simulink model "nms_sim_2D_cost"  (R2024b)
settings: Solver=ode15s  StartTime=0.0  StopTime=t_sim  MaxStep=dt_max  EnableMultiTasking=on
values from neighbouring files (symbols this model uses):
  a_BFSH = param_ctrl(35)*1    [setCtrlPar_optim_CPGreflex2001_2D.m]
  a_GAS = param_ctrl(37)*1    [setCtrlPar_optim_CPGreflex2001_2D.m]
  a_GLU = param_ctrl(31)*1    [setCtrlPar_optim_CPGreflex2001_2D.m]
  a_HAM = param_ctrl(33)*1    [setCtrlPar_optim_CPGreflex2001_2D.m]
  a_HFL = param_ctrl(32)*1    [setCtrlPar_optim_CPGreflex2001_2D.m]
  a_RF = param_ctrl(34)*1    [setCtrlPar_optim_CPGreflex2001_2D.m]
  a_SOL = param_ctrl(38)*1    [setCtrlPar_optim_CPGreflex2001_2D.m]
  a_TA = param_ctrl(39)*1    [setCtrlPar_optim_CPGreflex2001_2D.m]
  a_VAS = param_ctrl(36)*1    [setCtrlPar_optim_CPGreflex2001_2D.m]
  ai = param_ctrl(96)*2.0    [setCtrlPar_optim_CPGreflex2001_2D.m]
  b_BFSH = param_ctrl(52)*.51    [setCtrlPar_optim_CPGreflex2001_2D.m]
  b_BFSHGAS = param_ctrl(55)*.51    [setCtrlPar_optim_CPGreflex2001_2D.m]
  b_BFSHHAM = param_ctrl(54)*.51    [setCtrlPar_optim_CPGreflex2001_2D.m]
  b_BFSHVAS = param_ctrl(53)*.51    [setCtrlPar_optim_CPGreflex2001_2D.m]
  b_GAS = param_ctrl(59)*.51    [setCtrlPar_optim_CPGreflex2001_2D.m]
  b_GASBFSH = param_ctrl(60)*.51    [setCtrlPar_optim_CPGreflex2001_2D.m]
  b_GASSOL = param_ctrl(61)*.51    [setCtrlPar_optim_CPGreflex2001_2D.m]
  b_GLU = param_ctrl(40)*.51    [setCtrlPar_optim_CPGreflex2001_2D.m]
  b_GLUHAM = param_ctrl(42)*.51    [setCtrlPar_optim_CPGreflex2001_2D.m]
  b_GLUHFL = param_ctrl(41)*.51    [setCtrlPar_optim_CPGreflex2001_2D.m]
  b_HAM = param_ctrl(46)*.51    [setCtrlPar_optim_CPGreflex2001_2D.m]
  b_HAMBFSH = param_ctrl(48)*.51    [setCtrlPar_optim_CPGreflex2001_2D.m]
  b_HAMGLU = param_ctrl(47)*.51    [setCtrlPar_optim_CPGreflex2001_2D.m]
  b_HFL = param_ctrl(43)*.51    [setCtrlPar_optim_CPGreflex2001_2D.m]
  b_HFLGLU = param_ctrl(44)*.51    [setCtrlPar_optim_CPGreflex2001_2D.m]
  b_HFLRF = param_ctrl(45)*.51    [setCtrlPar_optim_CPGreflex2001_2D.m]
  b_RF = param_ctrl(49)*.51    [setCtrlPar_optim_CPGreflex2001_2D.m]
  b_RFHFL = param_ctrl(50)*.51    [setCtrlPar_optim_CPGreflex2001_2D.m]
  b_RFVAS = param_ctrl(51)*.51    [setCtrlPar_optim_CPGreflex2001_2D.m]
  b_SOL = param_ctrl(62)*.51    [setCtrlPar_optim_CPGreflex2001_2D.m]
  b_SOLGAS = param_ctrl(64)*.51    [setCtrlPar_optim_CPGreflex2001_2D.m]
  b_SOLTA = param_ctrl(63)*.51    [setCtrlPar_optim_CPGreflex2001_2D.m]
  b_TA = param_ctrl(65)*.51    [setCtrlPar_optim_CPGreflex2001_2D.m]
  b_TASOL = param_ctrl(66)*.51    [setCtrlPar_optim_CPGreflex2001_2D.m]
  b_VAS = param_ctrl(56)*.51    [setCtrlPar_optim_CPGreflex2001_2D.m]
  b_VASBFSH = param_ctrl(57)*.51    [setCtrlPar_optim_CPGreflex2001_2D.m]
  b_VASRF = param_ctrl(58)*.51    [setCtrlPar_optim_CPGreflex2001_2D.m]
  bias = param_ctrl(97)*2.5    [setCtrlPar_optim_CPGreflex2001_2D.m]
  c = 0.05    [nms_MS_2D_scaled.m]
  c_jointstop = 0.3 / (pi/180)    (= 17.1887338539)    [nms_MS_2D_scaled.m]
  D12_F = 0.16    *scaleL_JPhys    [nms_MechInit_2D_scaleSkel.m]
  D12_S = 0.2460	*sub_height    [nms_MechInit_2D_scaleSkel.m]
  D12_T = 0.2450  *sub_height    [nms_MechInit_2D_scaleSkel.m]
  D12y_F = 0.039  *sub_height    [nms_MechInit_2D_scaleSkel.m]
  D12z_HAT = 0.1    [nms_MS_2D_scaled.m]
  D13_F = 0.20    *scaleL_JPhys    [nms_MechInit_2D_scaleSkel.m]
  D1G_F = 0.14    *scaleL_JPhys    [nms_MechInit_2D_scaleSkel.m]
  D1G_HAT = 0.35  *scaleL_JPhys    [nms_MechInit_2D_scaleSkel.m]
  D1G_S = (0.3 - D12y_F/4)	*scaleL_JPhys    [nms_MechInit_2D_scaleSkel.m]
  D1G_T = (0.3 - D12y_F/4)	*scaleL_JPhys    [nms_MechInit_2D_scaleSkel.m]
  D1Gy_F = D12y_F*D1G_F/D12_F    (= 0.07)    [nms_MechInit_2D_scaleSkel.m]
  d_BFSH = param_ctrl(26)*1    [setCtrlPar_optim_CPGreflex2001_2D.m]
  d_GAS = param_ctrl(28)*1    [setCtrlPar_optim_CPGreflex2001_2D.m]
  d_GLU = param_ctrl(22)*1    [setCtrlPar_optim_CPGreflex2001_2D.m]
  d_HAM = param_ctrl(24)*1    [setCtrlPar_optim_CPGreflex2001_2D.m]
  d_HFL = param_ctrl(23)*1    [setCtrlPar_optim_CPGreflex2001_2D.m]
  d_RF = param_ctrl(25)*1    [setCtrlPar_optim_CPGreflex2001_2D.m]
  d_SOL = param_ctrl(29)*1    [setCtrlPar_optim_CPGreflex2001_2D.m]
  d_TA = param_ctrl(30)*1    [setCtrlPar_optim_CPGreflex2001_2D.m]
  d_VAS = param_ctrl(27)*1    [setCtrlPar_optim_CPGreflex2001_2D.m]
  DeltaThRef = 5e-3    (= 0.005)    [nms_MS_2D_scaled.m]
  dloptBFSH = 3.0    (= 3)    [setCtrlPar_optim_CPGreflex2001_2D.m]
  dloptGAS = 3.0    (= 3)    [setCtrlPar_optim_CPGreflex2001_2D.m]
  dloptGLU = 3.0    (= 3)    [setCtrlPar_optim_CPGreflex2001_2D.m]
  dloptHAM = 3.0    (= 3)    [setCtrlPar_optim_CPGreflex2001_2D.m]
  dloptHFL = 3.0    (= 3)    [setCtrlPar_optim_CPGreflex2001_2D.m]
  dloptRF = 3.0    (= 3)    [setCtrlPar_optim_CPGreflex2001_2D.m]
  dloptSOL = 3.0    (= 3)    [setCtrlPar_optim_CPGreflex2001_2D.m]
  dloptTA = 3.0    (= 3)    [setCtrlPar_optim_CPGreflex2001_2D.m]
  dloptVAS = 3.0    (= 3)    [setCtrlPar_optim_CPGreflex2001_2D.m]
  ec_BFSH = param_ctrl(80)*0.15    [setCtrlPar_optim_CPGreflex2001_2D.m]
  ec_GAS = param_ctrl(82)*0.15    [setCtrlPar_optim_CPGreflex2001_2D.m]
  ec_GLU = param_ctrl(76)*0.15    [setCtrlPar_optim_CPGreflex2001_2D.m]
  ec_HAM = param_ctrl(78)*0.15    [setCtrlPar_optim_CPGreflex2001_2D.m]
  ec_HFL = param_ctrl(77)*0.15    [setCtrlPar_optim_CPGreflex2001_2D.m]
  ec_RF = param_ctrl(79)*0.15    [setCtrlPar_optim_CPGreflex2001_2D.m]
  ec_TA = param_ctrl(84)*0.15    [setCtrlPar_optim_CPGreflex2001_2D.m]
  ec_VAS = param_ctrl(81)*0.15    [setCtrlPar_optim_CPGreflex2001_2D.m]
  eref = 0.04    [nms_MS_2D_scaled.m]
  eref_GAS = 0.1    [nms_MS_2D_scaled.m]
  eref_SOL = 0.1    [nms_MS_2D_scaled.m]
  es_BFSH = param_ctrl(89)*0.15    [setCtrlPar_optim_CPGreflex2001_2D.m]
  es_GAS = param_ctrl(91)*0.15    [setCtrlPar_optim_CPGreflex2001_2D.m]
  es_GLU = param_ctrl(85)*0.15    [setCtrlPar_optim_CPGreflex2001_2D.m]
  es_HAM = param_ctrl(87)*0.15    [setCtrlPar_optim_CPGreflex2001_2D.m]
  es_HFL = param_ctrl(86)*0.15    [setCtrlPar_optim_CPGreflex2001_2D.m]
  es_RF = param_ctrl(88)*0.15    [setCtrlPar_optim_CPGreflex2001_2D.m]
  es_TA = param_ctrl(93)*0.15    [setCtrlPar_optim_CPGreflex2001_2D.m]
  es_VAS = param_ctrl(90)*0.15    [setCtrlPar_optim_CPGreflex2001_2D.m]
  FmaxBFSH = 350    [nms_MS_2D_scaled.m]
  FmaxGAS = 2000    [nms_MS_2D_scaled.m]
  FmaxGLU = 4000    [nms_MS_2D_scaled.m]
  FmaxHAM = 2000    [nms_MS_2D_scaled.m]
  FmaxHFL = 2000    [nms_MS_2D_scaled.m]
  FmaxRF = 850    [nms_MS_2D_scaled.m]
  FmaxSOL = 4000    [nms_MS_2D_scaled.m]
  FmaxTA = 800    [nms_MS_2D_scaled.m]
  FmaxVAS = 5000    [nms_MS_2D_scaled.m]
  g = 9.81    [nms_MS_2D_scaled.m]
  gamma_4 = param_ctrl(11) * 1.7    [setCtrlPar_optim_CPGreflexsynergy2023_2D.m]
  h_BFSH = param_ctrl(71)*.1    [setCtrlPar_optim_CPGreflex2001_2D.m]
  h_GAS = param_ctrl(73)*.1    [setCtrlPar_optim_CPGreflex2001_2D.m]
  h_GLU = param_ctrl(67)*.1    [setCtrlPar_optim_CPGreflex2001_2D.m]
  h_HAM = param_ctrl(69)*.1    [setCtrlPar_optim_CPGreflex2001_2D.m]
  h_HFL = param_ctrl(68)*.1    [setCtrlPar_optim_CPGreflex2001_2D.m]
  h_RF = param_ctrl(70)*.1    [setCtrlPar_optim_CPGreflex2001_2D.m]
  h_SOL = param_ctrl(74)*.1    [setCtrlPar_optim_CPGreflex2001_2D.m]
  h_TA = param_ctrl(75)*.1    [setCtrlPar_optim_CPGreflex2001_2D.m]
  h_VAS = param_ctrl(72)*.1    [setCtrlPar_optim_CPGreflex2001_2D.m]
  HLCtrlPar = [theta_tgt l_clr alpha_tgt alpha_cd alpha_cv]    [setCtrlPar_optim_reflex2015_2D.m]
  In_F = 0.005    *scaleM*scaleL_JPhys^2    [nms_MechInit_2D_scaleSkel.m]
  In_HAT = 2.5    *scaleM*scaleL_JPhys^2    [nms_MechInit_2D_scaleSkel.m]
  In_S = 0.05     *scaleM*scaleL_JPhys^2    [nms_MechInit_2D_scaleSkel.m]
  In_T = 0.15     *scaleM*scaleL_JPhys^2    [nms_MechInit_2D_scaleSkel.m]
  init_exc = 0.01    [setInitPar_optim_2D.m]
  init_fm = 0.01    [setInitPar_optim_2D.m]
  init_lce = 1    [setInitPar_optim_2D.m]
  init_LCPG = param_ctrl(12) * 0.01    [setCtrlPar_optim_CPGreflexsynergy2023_2D.m]
  init_LStance = 1    [setInitPar_optim_2D.m]
  init_N1 = osc_signal1(phi_off_osc_ind)    [setCtrlPar_optim_CPGreflex2001_2D.m]
  ... (+441 more)
undefined symbols (not defined in the file or in its folder): cost_act_exponent, cost_v_tgt, flag_controller, Newton, nStep_obj, nStep_startKin, Raphson, sgn, SSW_kin, terrain_slope_angle, v_plateS1, X, Y, Z
libraries: nesl_utility x94, sm_lib x90, simulink x28, simulink_extras x12
(part 2 of 20)

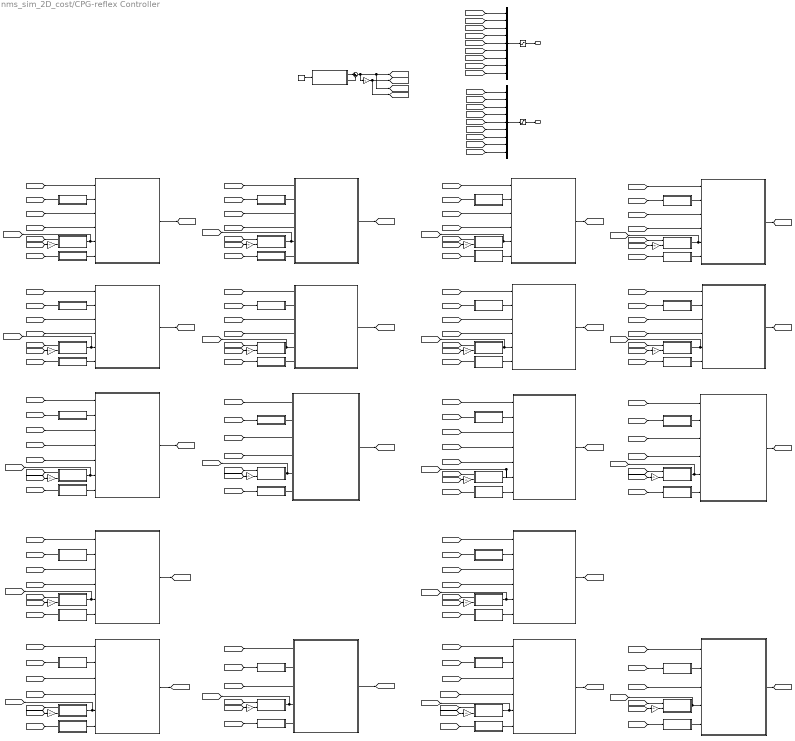
== system nms_sim_2D_cost/CPG-reflex Controller ==
  note: GLU αMN
  note: HAM αMN
  note: HFL αMN
  note: RF αMN
  note: BFSH αMN
  note: VAS αMN
  note: SOL αMN
  note: TA αMN
  note: GAS αMN
  note: Rhythm Generator
  note: HAM αMN
  note: GAS αMN
  note: SOL αMN
  note: VAS αMN
  note: TA αMN
  note: BFSH αMN
  note: GLU αMN
  note: HFL αMN
  note: RF αMN
  Alpha moto-neuron : Subsystem
  Alpha moto-neuron1 : Subsystem
  Alpha moto-neuron18 : Subsystem
  Alpha moto-neuron19 : Subsystem
  Alpha moto-neuron2 : Subsystem
  Alpha moto-neuron20 : Subsystem
  Alpha moto-neuron21 : Subsystem
  Alpha moto-neuron22 : Subsystem
  Alpha moto-neuron23 : Subsystem
  Alpha moto-neuron24 : Subsystem
  Alpha moto-neuron25 : Subsystem
  Alpha moto-neuron26 : Subsystem
  Alpha moto-neuron3 : Subsystem
  Alpha moto-neuron4 : Subsystem
  Alpha moto-neuron5 : Subsystem
  Alpha moto-neuron6 : Subsystem
  Alpha moto-neuron7 : Subsystem
  Alpha moto-neuron8 : Subsystem
  CPG : Subsystem
  FB VAS : Subsystem
  FB VAS2 : Subsystem
  Feedback HAM : Subsystem
  Feedback HAM2 : Subsystem
  Gain1 : Gain  Gain=-1
  Golgi tendon organ BFSH : Subsystem
  Golgi tendon organ BFSH2 : Subsystem
  Golgi tendon organ GAS : Subsystem
  Golgi tendon organ GAS2 : Subsystem
  Golgi tendon organ GLU : Subsystem
  Golgi tendon organ GLU2 : Subsystem
  Golgi tendon organ HAM : Subsystem
  Golgi tendon organ HAM2 : Subsystem
  Golgi tendon organ HFL : Subsystem
  Golgi tendon organ HFL2 : Subsystem
  Golgi tendon organ RF : Subsystem
  Golgi tendon organ RF2 : Subsystem
  Golgi tendon organ SOL : Subsystem
  Golgi tendon organ SOL2 : Subsystem
  Golgi tendon organ TA : Subsystem
  Golgi tendon organ TA2 : Subsystem
  Golgi tendon organ VAS : Subsystem
  Golgi tendon organ VAS2 : Subsystem
  L HFL Muscle Spindles1 : Gain  Gain=loptBFSH/dloptBFSH
  L HFL Muscle Spindles10 : Gain  Gain=loptHAM/dloptHAM
  L HFL Muscle Spindles11 : Gain  Gain=loptGLU/dloptGLU
  L HFL Muscle Spindles12 : Gain  Gain=loptGAS/dloptGAS
  L HFL Muscle Spindles13 : Gain  Gain=loptSOL/dloptSOL
  L HFL Muscle Spindles14 : Gain  Gain=loptTA/dloptTA
  L HFL Muscle Spindles15 : Gain  Gain=loptVAS/dloptVAS
  L HFL Muscle Spindles16 : Gain  Gain=loptRF/dloptRF
  L HFL Muscle Spindles17 : Gain  Gain=loptHFL/dloptHFL
  L HFL Muscle Spindles19 : Gain  Gain=loptHAM/dloptHAM
  L HFL Muscle Spindles2 : Gain  Gain=loptGLU/dloptGLU
  L HFL Muscle Spindles3 : Gain  Gain=loptGAS/dloptGAS
  L HFL Muscle Spindles4 : Gain  Gain=loptSOL/dloptSOL
  L HFL Muscle Spindles5 : Gain  Gain=loptTA/dloptTA
  L HFL Muscle Spindles6 : Gain  Gain=loptVAS/dloptVAS
  L HFL Muscle Spindles7 : Gain  Gain=loptRF/dloptRF
  L HFL Muscle Spindles8 : Gain  Gain=loptHFL/dloptHFL
  L HFL Muscle Spindles9 : Gain  Gain=loptBFSH/dloptBFSH
  Muscle Spindle BFSH : Subsystem
  Muscle Spindle BFSH2 : Subsystem
  Muscle Spindle GAS : Subsystem
  Muscle Spindle GAS2 : Subsystem
  Muscle Spindle GLU : Subsystem
  Muscle Spindle GLU2 : Subsystem
  Muscle Spindle HAM : Subsystem
  Muscle Spindle HAM2 : Subsystem
  Muscle Spindle HFL : Subsystem
  Muscle Spindle HFL2 : Subsystem
  Muscle Spindle RF : Subsystem
  Muscle Spindle RF2 : Subsystem
  Muscle Spindle SOL : Subsystem
  Muscle Spindle SOL2 : Subsystem
  Muscle Spindle TA : Subsystem
  Muscle Spindle TA2 : Subsystem
  Muscle Spindle VAS : Subsystem
  Muscle Spindle VAS2 : Subsystem
  Mux2 : Mux  Inputs=9
  Mux3 : Mux  Inputs=9
  Saturation2 : Saturate  UpperLimit=1  LowerLimit=0.01
  Saturation3 : Saturate  UpperLimit=1  LowerLimit=0.01
  Sum1 : Sum  Inputs=|+-
  Zero1 : Constant  Value=0  OutDataTypeStr=Inherit: Inherit via back propagation
  feedback : Subsystem
  feedback BFSH : Subsystem
  feedback BFSH2 : Subsystem
  feedback HFL : Subsystem
  feedback HFL2 : Subsystem
  feedback RF : Subsystem
  feedback RF2 : Subsystem
  feedback SOL : Subsystem
  feedback SOL2 : Subsystem
  feedback TA : Subsystem
  feedback TA2 : Subsystem
  feedback2 : Subsystem
  feedbackGAS : Subsystem
  feedbackGAS2 : Subsystem
  LExc : Outport
  RExc : Outport  Port=2
  wires:
  [d_LVceGLU] -> L HFL Muscle Spindles2/1
  [d_LLceGLU] -> Muscle Spindle GLU/1(Lce)
  [d_LFmGLU] -> Golgi tendon organ GLU/1(Fm)
  [d_LStance] -> feedback/1(LStance)
  [Lrhythm_ext] -> Alpha moto-neuron/1(rhythm_ext)
  Golgi tendon organ GLU/1(Gm) -> Alpha moto-neuron/2(GGLU)
  Muscle Spindle GLU/1(Sm) -> [LMSGLU], Alpha moto-neuron/5(SGLU)
  feedback/1(Feedback) -> Alpha moto-neuron/6(Feedback)
  Feedback HAM/1(FBHAM) -> Alpha moto-neuron1/6(FBHAM)
  [d_LVceHAM] -> L HFL Muscle Spindles19/1
  [d_LStance] -> Feedback HAM/1(LStance)
  [d_LFmHAM] -> Golgi tendon organ HAM/1(Fm)
  [d_LLceHAM] -> Muscle Spindle HAM/1(Lce)
  [d_LLceRF] -> Muscle Spindle RF/1(Lce)
  [d_LFmRF] -> Golgi tendon organ RF/1(FRF)
  [d_LStance] -> feedback RF/1(LStance)
  [d_LVceRF] -> L HFL Muscle Spindles7/1
  [d_LStance] -> feedback HFL/1(LStance)
  [d_LFmHFL] -> Golgi tendon organ HFL/1(FmHFL)
  [d_LLceHFL] -> Muscle Spindle HFL/1(Lce)
  [d_LVceHFL] -> L HFL Muscle Spindles8/1
  [d_LVceVAS] -> L HFL Muscle Spindles6/1
  [d_LStance] -> FB VAS/1(LStance)
  [d_LFmVAS] -> Golgi tendon organ VAS/1(FmVAS)
  [d_LLceVAS] -> Muscle Spindle VAS/1(Lce)
  [d_LLceBFSH] -> Muscle Spindle BFSH/1(Lce)
  [Lrhythm_flex] -> Alpha moto-neuron4/1(rhythm_ext)
  Golgi tendon organ BFSH/1(GBFSH) -> Alpha moto-neuron4/2(GBFSH)
  [d_LFmBFSH] -> Golgi tendon organ BFSH/1(FBFSH)
  [d_LStance] -> feedback BFSH/1(LStance)
  [d_LVceBFSH] -> L HFL Muscle Spindles1/1
  feedback BFSH/1(FBBFSH) -> Alpha moto-neuron4/7(FBBFSH)
  feedback SOL/1(FB SOL) -> Alpha moto-neuron6/6(FB SOL)
  [d_LVceSOL] -> L HFL Muscle Spindles4/1
  [d_LStance] -> feedback SOL/1(LStance)
  [d_LFmSOL] -> Golgi tendon organ SOL/1(FmSOL)
  Muscle Spindle SOL/1(Sm) -> [LMSSOL], Alpha moto-neuron6/5(SSOL)
  Golgi tendon organ SOL/1(GSOL) -> Alpha moto-neuron6/2(GSOL)
  [Lrhythm_ext] -> Alpha moto-neuron6/1(rhythm_ext)
  [d_LLceSOL] -> Muscle Spindle SOL/1(Lce)
  [d_LLceTA] -> Muscle Spindle TA/1(Lce)
  [d_LFmTA] -> Golgi tendon organ TA/1(FTA)
  [d_LStance] -> feedback TA/1(LStance)
  [d_LVceTA] -> L HFL Muscle Spindles5/1
  [d_LLceGAS] -> Muscle Spindle GAS/1(Lce)
  [Lrhythm_ext] -> Alpha moto-neuron8/1(rhythm_ext)
  Golgi tendon organ GAS/1(GGAS) -> Alpha moto-neuron8/2(GGAS)
  [d_LFmGAS] -> Golgi tendon organ GAS/1(FmGAS)
  [d_LStance] -> feedbackGAS/1(LStance)
  [d_LVceGAS] -> L HFL Muscle Spindles3/1
  feedbackGAS/1(FB GAS) -> Alpha moto-neuron8/6(FBGAS)
  Muscle Spindle GAS/1(Sm) -> Alpha moto-neuron8/5(SGAS), [LMSGAS]
  Muscle Spindle BFSH/1(Sm) -> [LMSBFSH], Alpha moto-neuron4/6(SBFSH)
  [LMSHFL] -> Alpha moto-neuron/3(LMSHFL)
  [LMSHAM] -> Alpha moto-neuron/4(LMSHAM)
  Alpha moto-neuron/1(LExcGLU) -> [LExcAMN_GLU]
  Alpha moto-neuron2/1(LExcHFL) -> [LExcAMN_HFL]
  [LMSVAS] -> Alpha moto-neuron4/3(LMSVAS)
  [LMSHAM] -> Alpha moto-neuron4/5(LMSHAM)
  [LMSGAS] -> Alpha moto-neuron4/4(LMSGAS)
  [LMSBFSH] -> Alpha moto-neuron8/3(LMSBFSH)
  [LMSSOL] -> Alpha moto-neuron8/4(LMSSOL)
  [LMSTA] -> Alpha moto-neuron6/3(LMSTA)
  [LMSGAS] -> Alpha moto-neuron6/4(LMSGAS)
  Alpha moto-neuron1/1(LExcHAM) -> [LExcAMN_HAM]
  Alpha moto-neuron4/1(LExcBFSH) -> [LExcAMN_BFSH]
  Alpha moto-neuron8/1(LExcGAS) -> [LExcAMN_GAS]
  Alpha moto-neuron6/1(LExcSOL) -> [LExcAMN_SOL]
  Alpha moto-neuron7/1(LExcTA) -> [LExcAMN_TA]
  Alpha moto-neuron5/1(LExcVAS) -> [LExcAMN_VAS]
  Alpha moto-neuron3/1(LExcRF) -> [LExcAMN_RF]
  [Lrhythm_flex] -> Alpha moto-neuron1/1(rhythm_ext)
  Golgi tendon organ HAM/1(Gm) -> Alpha moto-neuron1/2(GHAM)
  [LMSBFSH] -> Alpha moto-neuron1/4(LMSBFSH)
  Muscle Spindle HAM/1(Sm) -> Alpha moto-neuron1/5(SHAM), [LMSHAM]
  [LMSGLU] -> Alpha moto-neuron1/3(LMSGLU)
  Muscle Spindle TA/1(Sm) -> [LMSTA], Alpha moto-neuron7/4(STA)
  [LMSSOL] -> Alpha moto-neuron7/3(LMSSOL)
  feedback TA/1(FB TA) -> Alpha moto-neuron7/5(FB TA)  "fb"
  Golgi tendon organ TA/1(GTA) -> Alpha moto-neuron7/2(GTA)
  [Lrhythm_flex] -> Alpha moto-neuron7/1(rhythm_flex)
  [LMSRF] -> Alpha moto-neuron5/4(LMSRF)
  [LMSBFSH] -> Alpha moto-neuron5/3(LMSBFSH)
  Muscle Spindle VAS/1(Sm) -> [LMSVAS], Alpha moto-neuron5/5(SVAS)
  FB VAS/1(FBVAS) -> Alpha moto-neuron5/6(FBVAS)
  Golgi tendon organ VAS/1(GVAS) -> Alpha moto-neuron5/2(GVAS)
  [Lrhythm_ext] -> Alpha moto-neuron5/1(rhythm_flex)
  [Lrhythm_ext] -> Alpha moto-neuron3/1(rhythm_flex)
  Golgi tendon organ RF/1(GRF) -> Alpha moto-neuron3/2(GRF)  "golgi"
  feedback RF/1(Feedback) -> Alpha moto-neuron3/6(FBRF)
  Muscle Spindle RF/1(Sm) -> [LMSRF], Alpha moto-neuron3/5(SRF)
  [LMSHFL] -> Alpha moto-neuron3/3(LMSHFL)
  [LMSVAS] -> Alpha moto-neuron3/4(LMSVAS)
  [LMSRF] -> Alpha moto-neuron2/4(LMSRF)
  [LMSGLU] -> Alpha moto-neuron2/3(LMSGLU)
  Muscle Spindle HFL/1(Sm) -> [LMSHFL], Alpha moto-neuron2/5(SHFL)
  feedback HFL/1(FBHFL) -> Alpha moto-neuron2/6(FBHFL)
  Golgi tendon organ HFL/1(GHFL) -> Alpha moto-neuron2/2(GHFL)
  [Lrhythm_flex] -> Alpha moto-neuron2/1(rhythm_flex)
  L HFL Muscle Spindles2/1 -> Muscle Spindle GLU/2(Vce)
  L HFL Muscle Spindles19/1 -> Muscle Spindle HAM/2(Vce)
  L HFL Muscle Spindles1/1 -> Muscle Spindle BFSH/2(Vce)
  L HFL Muscle Spindles3/1 -> Muscle Spindle GAS/2(Vce)
  L HFL Muscle Spindles4/1 -> Muscle Spindle SOL/2(Vce)
  L HFL Muscle Spindles5/1 -> Muscle Spindle TA/2(Vce)
  L HFL Muscle Spindles6/1 -> Muscle Spindle VAS/2(Vce)
  L HFL Muscle Spindles7/1 -> Muscle Spindle RF/2(Vce)
  L HFL Muscle Spindles8/1 -> Muscle Spindle HFL/2(Vce)
  [RExcAMN_SOL] -> Mux3/8
  [RExcAMN_RF] -> Mux3/4
  CPG/2(Outport1) -> Sum1/2
  Zero1/1 -> CPG/1(FB)
  [RExcAMN_GLU] -> Mux3/2
  [RExcAMN_HFL] -> Mux3/1
  [LExcAMN_GAS] -> Mux2/7
  [LExcAMN_HFL] -> Mux2/1
  [LExcAMN_SOL] -> Mux2/8
  Sum1/1 -> Gain1/1, [Rrhythm_flex], [Lrhythm_ext]
  [RExcAMN_VAS] -> Mux3/5
  [LExcAMN_RF] -> Mux2/4
  [LExcAMN_HAM] -> Mux2/3
  [RExcAMN_BFSH] -> Mux3/6
  [LExcAMN_BFSH] -> Mux2/6
  Saturation2/1 -> LExc/1
  [RExcAMN_TA] -> Mux3/9
  Saturation3/1 -> RExc/1
  [LExcAMN_VAS] -> Mux2/5
  CPG/1(Outport) -> Sum1/1
  [RExcAMN_HAM] -> Mux3/3
  [LExcAMN_TA] -> Mux2/9
  [RExcAMN_GAS] -> Mux3/7
  Gain1/1 -> [Rrhythm_ext], [Lrhythm_flex]
  Mux2/1 -> Saturation2/1
  Mux3/1 -> Saturation3/1
  [LExcAMN_GLU] -> Mux2/2
  Golgi tendon organ TA2/1(GTA) -> Alpha moto-neuron24/2(GTA)  "golgi"
  L HFL Muscle Spindles9/1 -> Muscle Spindle BFSH2/2(Vce)
  [RMSVAS] -> Alpha moto-neuron20/4(LMSVAS)  "msVAS"
  [d_RLceHAM] -> Muscle Spindle HAM2/1(Lce)
  Alpha moto-neuron19/1(RExcHFL) -> [RExcAMN_HFL]
  Golgi tendon organ SOL2/1(GSOL) -> Alpha moto-neuron23/2(GSOL)  "golgi"
  Alpha moto-neuron23/1(RExcSOL) -> [RExcAMN_SOL]
  L HFL Muscle Spindles17/1 -> Muscle Spindle HFL2/2(Vce)
  [d_RStance] -> FB VAS2/1(RStance)
  [RMSRF] -> Alpha moto-neuron22/4(LMSRF)  "msrf"
  [d_RStance] -> feedback TA2/1(RStance)
  Muscle Spindle HAM2/1(Sm) -> [RMSHAM], Alpha moto-neuron18/5(SHAM)  "msham"
  [d_RFmBFSH] -> Golgi tendon organ BFSH2/1(FBFSH)
  Golgi tendon organ GAS2/1(GGAS) -> Alpha moto-neuron25/2(GGAS)  "golgi"
  Muscle Spindle VAS2/1(Sm) -> Alpha moto-neuron22/5(SVAS), [RMSVAS]  "ms"
  [d_RFmGAS] -> Golgi tendon organ GAS2/1(FmGAS)
  [RMSBFSH] -> Alpha moto-neuron22/3(LMSBFSH)  "msbfsh"
  [Rrhythm_flex] -> Alpha moto-neuron21/1(rhythm_ext)  "rhythm"
  [d_RFmSOL] -> Golgi tendon organ SOL2/1(FmSOL)
  [RMSGLU] -> Alpha moto-neuron19/3(LMSGLU)  "MSGLU"
  [d_RVceSOL] -> L HFL Muscle Spindles13/1
  [RMSGLU] -> Alpha moto-neuron18/3(LMSGLU)  "msglu"
  [d_RFmTA] -> Golgi tendon organ TA2/1(FTA)
  Alpha moto-neuron18/1(RExcHAM) -> [RExcAMN_HAM]
  Golgi tendon organ GLU2/1(GGLU) -> Alpha moto-neuron26/2(GGLU)  "msglu"
  feedback BFSH2/1(FBBFSH) -> Alpha moto-neuron21/7(FBBFSH)  "fb"
  Alpha moto-neuron21/1(RExcBFSH) -> [RExcAMN_BFSH]
  [d_RFmGLU] -> Golgi tendon organ GLU2/1(Fm)
  Golgi tendon organ HFL2/1(GHFL) -> Alpha moto-neuron19/2(GHFL)  "golgi tendon"
  [d_RStance] -> feedbackGAS2/1(RStance)
  [RMSGAS] -> Alpha moto-neuron23/4(LMSGAS)  "msgas"
  [d_RVceBFSH] -> L HFL Muscle Spindles9/1
  [RMSBFSH] -> Alpha moto-neuron18/4(LMSBFSH)  "msbfsh"
  [d_RVceGLU] -> L HFL Muscle Spindles11/1
  [d_RStance] -> feedback2/1(RStance)
  Muscle Spindle TA2/1(Sm) -> [RMSTA], Alpha moto-neuron24/4(STA)  "ms"
  [d_RVceGAS] -> L HFL Muscle Spindles12/1
  [d_RFmHAM] -> Golgi tendon organ HAM2/1(FHAM)
  Alpha moto-neuron25/1(RExcGAS) -> [RExcAMN_GAS]
  Alpha moto-neuron20/1(RExcRF) -> [RExcAMN_RF]
  [d_RStance] -> Feedback HAM2/1(RStance)
  L HFL Muscle Spindles14/1 -> Muscle Spindle TA2/2(Vce)
  [d_RVceHAM] -> L HFL Muscle Spindles10/1
  [RMSHFL] -> Alpha moto-neuron20/3(LMSHFL)  "msHFL"
  Alpha moto-neuron24/1(RExcTA) -> [RExcAMN_TA]
  [d_RVceTA] -> L HFL Muscle Spindles14/1
  [d_RVceHFL] -> L HFL Muscle Spindles17/1
  [d_RVceRF] -> L HFL Muscle Spindles16/1
  L HFL Muscle Spindles10/1 -> Muscle Spindle HAM2/2(Vce)
  L HFL Muscle Spindles11/1 -> Muscle Spindle GLU2/2(Vce)
  [Rrhythm_ext] -> Alpha moto-neuron25/1(rhythm_ext)  "rhythm"
  [Rrhythm_ext] -> Alpha moto-neuron20/1(rhythm_flex)  "rhythm"
  Alpha moto-neuron26/1(RExcGLU) -> [RExcAMN_GLU]
  [d_RStance] -> feedback BFSH2/1(RStance)
  [d_RFmHFL] -> Golgi tendon organ HFL2/1(FmHFL)
  Muscle Spindle GLU2/1(Sm) -> [RMSGLU], Alpha moto-neuron26/5(SGLU)  "msglu"
  [d_RLceGLU] -> Muscle Spindle GLU2/1(Lce)
  Muscle Spindle HFL2/1(Sm) -> [RMSHFL], Alpha moto-neuron19/5(SHFL)  "Muscle spindle"
  Muscle Spindle BFSH2/1(Sm) -> Alpha moto-neuron21/6(SBFSH), [RMSBFSH]  "msBFSH"
  [d_RFmVAS] -> Golgi tendon organ VAS2/1(FmVAS)
  L HFL Muscle Spindles15/1 -> Muscle Spindle VAS2/2(Vce)
  feedback2/1(Feedback) -> Alpha moto-neuron26/6(Feedback)  "fb"
  [RMSHAM] -> Alpha moto-neuron26/4(LMSHAM)  "msham"
  [RMSSOL] -> Alpha moto-neuron25/4(LMSSOL)  "mssol"
  [d_RLceGAS] -> Muscle Spindle GAS2/1(Lce)
  feedbackGAS2/1(FB GAS) -> Alpha moto-neuron25/6(FBGAS)  "fb"
  L HFL Muscle Spindles16/1 -> Muscle Spindle RF2/2(Vce)
  Muscle Spindle GAS2/1(Sm) -> [RMSGAS], Alpha moto-neuron25/5(SGAS)  "msgas"
  [Rrhythm_ext] -> Alpha moto-neuron22/1(rhythm_flex)  "rhythm"
  [d_RLceHFL] -> Muscle Spindle HFL2/1(Lce)
  [d_RStance] -> feedback SOL2/1(RStance)
  L HFL Muscle Spindles12/1 -> Muscle Spindle GAS2/2(Vce)
  [d_RFmRF] -> Golgi tendon organ RF2/1(FRF)
  Golgi tendon organ HAM2/1(GHAM) -> Alpha moto-neuron18/2(GHAM)  "golgi"
  [d_RLceVAS] -> Muscle Spindle VAS2/1(Lce)
  Muscle Spindle SOL2/1(Sm) -> Alpha moto-neuron23/5(SSOL), [RMSSOL]  "mssol"
  [d_RLceTA] -> Muscle Spindle TA2/1(Lce)
  [Rrhythm_flex] -> Alpha moto-neuron19/1(rhythm_flex)  "rhythm"
  Golgi tendon organ VAS2/1(GVAS) -> Alpha moto-neuron22/2(GVAS)  "golgi"
  Golgi tendon organ BFSH2/1(GBFSH) -> Alpha moto-neuron21/2(GBFSH)  "golgi"
  L HFL Muscle Spindles13/1 -> Muscle Spindle SOL2/2(Vce)
  [RMSBFSH] -> Alpha moto-neuron25/3(LMSBFSH)  "msbfsh"
  Muscle Spindle RF2/1(Sm) -> [RMSRF], Alpha moto-neuron20/5(SRF)  "msRF"
  Golgi tendon organ RF2/1(GRF) -> Alpha moto-neuron20/2(GRF)  "golgi"
  Alpha moto-neuron22/1(RExcVAS) -> [RExcAMN_VAS]
  feedback TA2/1(FB TA) -> Alpha moto-neuron24/5(FB TA)  "fb"
  [d_RLceSOL] -> Muscle Spindle SOL2/1(Lce)
  [d_RStance] -> feedback RF2/1(RStance)
  [Rrhythm_flex] -> Alpha moto-neuron18/1(rhythm_ext)  "rhythm"
  feedback SOL2/1(FB SOL) -> Alpha moto-neuron23/6(FB SOL)  "fb"
  feedback RF2/1(Feedback) -> Alpha moto-neuron20/6(FBRF)  "fb"
  [RMSHAM] -> Alpha moto-neuron21/5(LMSHAM)  "msham"
  [d_RVceVAS] -> L HFL Muscle Spindles15/1
  [RMSHFL] -> Alpha moto-neuron26/3(LMSHFL)  "mshfl"
  [Rrhythm_flex] -> Alpha moto-neuron24/1(rhythm_flex)  "rhythm"
  [Rrhythm_ext] -> Alpha moto-neuron26/1(rhythm_ext)  "rhythm"
  [d_RStance] -> feedback HFL2/1(RStance)
  [RMSRF] -> Alpha moto-neuron19/4(LMSRF)  "MSRF"
  FB VAS2/1(FBVAS) -> Alpha moto-neuron22/6(FBVAS)  "stance"
  [RMSSOL] -> Alpha moto-neuron24/3(LMSSOL)  "mssol"
  [Rrhythm_ext] -> Alpha moto-neuron23/1(rhythm_ext)  "rhythm"
  [d_RLceRF] -> Muscle Spindle RF2/1(Lce)
  [RMSVAS] -> Alpha moto-neuron21/3(LMSVAS)  "MSVAS"
  Feedback HAM2/1(FBHAM) -> Alpha moto-neuron18/6(FBHAM)  "fb"
  [RMSTA] -> Alpha moto-neuron23/3(LMSTA)  "msta"
  feedback HFL2/1(FBHFL) -> Alpha moto-neuron19/6(FBHFL)  "Stance"
  [d_RLceBFSH] -> Muscle Spindle BFSH2/1(Lce)
  [RMSGAS] -> Alpha moto-neuron21/4(LMSGAS)  "msGAS"

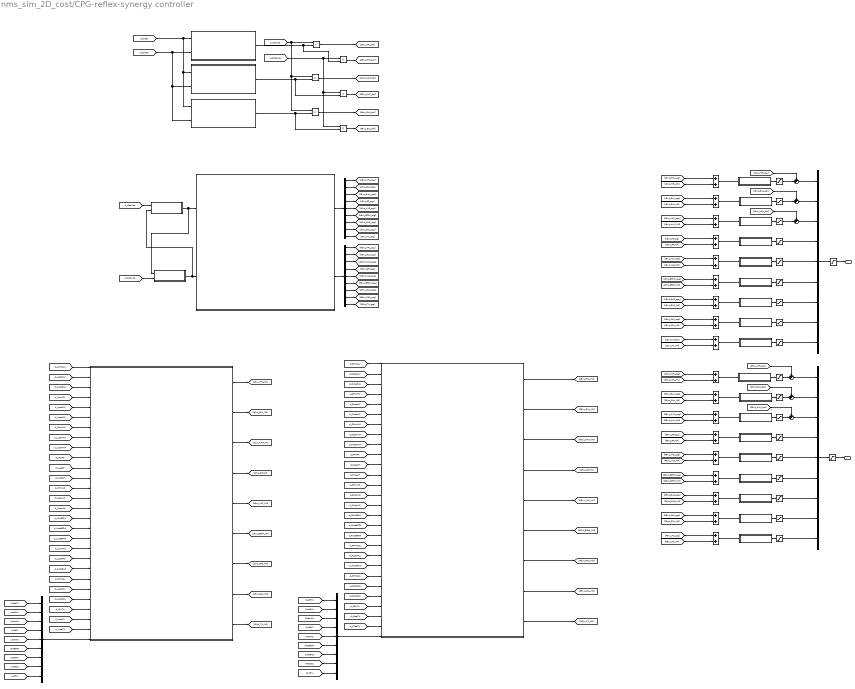
== system nms_sim_2D_cost/CPG-reflex-synergy controller ==
  note: BALANCE CONTROLLER
  note: CPG CONTROLLER
  note: REFLEX CONTROLLER
  Balance Control System GLU : Subsystem
  Balance Control System HAM : Subsystem
  Balance Control System HFL : Subsystem
  Central Pattern Generator : Subsystem
  Demux : Demux  Outputs=9
  Demux1 : Demux  Outputs=9
  MN : Subsystem
  MN1 : Subsystem
  MN10 : Subsystem
  MN11 : Subsystem
  MN12 : Subsystem
  MN13 : Subsystem
  MN14 : Subsystem
  MN15 : Subsystem
  MN16 : Subsystem
  MN17 : Subsystem
  MN2 : Subsystem
  MN3 : Subsystem
  MN4 : Subsystem
  MN5 : Subsystem
  MN6 : Subsystem
  MN7 : Subsystem
  MN8 : Subsystem
  MN9 : Subsystem
  Mux{,1..3} (4 alike) : Mux  Inputs=9
  Product{,1..5} (6 alike) : Product
  Reflexes1 : Subsystem
  Reflexes2 : Subsystem
  Saturation{1,18,44..61} (20 alike) : Saturate  UpperLimit=1  LowerLimit=0.01
  Sum{,2,4,7,19,21} (6 alike) : Sum  Inputs=++|
  Sum{1,3,5..6,8..18,20,22..23} (18 alike) : Sum
  phi left3 : Subsystem
  phi right : Subsystem
  LExc : Outport
  RExc : Outport  Port=2
  wires:
  [d_LStance] -> Product/1, Product2/1, Product4/1
  Balance Control System HFL/1(ubalance) -> Product/2, Product1/2
  [d_RStance] -> Product5/1, Product3/1, Product1/1
  Demux/1 -> [LExc_HFL_cpg]
  Demux/2 -> [LExc_GLU_cpg]
  Demux/3 -> [LExc_HAM_cpg]
  Demux/4 -> [LExc_RF_cpg]
  Demux/5 -> [LExc_VAS_cpg]
  Demux/6 -> [LExc_BFSH_cpg]
  Demux/7 -> [LExc_GAS_cpg]
  Demux/8 -> [LExc_SOL_cpg]
  Demux/9 -> [LExc_TA_cpg]
  Demux1/9 -> [RExc_TA_cpg]
  Demux1/8 -> [RExc_SOL_cpg]
  Demux1/7 -> [RExc_GAS_cpg]
  Demux1/6 -> [RExc_BFSH_cpg]
  Demux1/5 -> [RExc_VAS_cpg]
  Demux1/4 -> [RExc_RF_cpg]
  Demux1/3 -> [RExc_HAM_cpg]
  Demux1/2 -> [RExc_GLU_cpg]
  Demux1/1 -> [RExc_HFL_cpg]
  Saturation18/1 -> LExc/1
  Mux/1 -> Saturation18/1
  Saturation1/1 -> RExc/1
  Central Pattern Generator/1(Outport) -> Demux/1
  Central Pattern Generator/2(Outport1) -> Demux1/1
  [d_LFmGLU] -> Reflexes2/1(FmGLU)
  [d_LLceGLU] -> Reflexes2/2(LceGLU)
  [d_LVceGLU] -> Reflexes2/3(VceGLU)
  [d_LFmHFL] -> Reflexes2/4(FmHFL)
  [d_LLceHFL] -> Reflexes2/5(LceHFL)
  [d_LVceHFL] -> Reflexes2/6(VceHFL)
  [d_LFmHAM] -> Reflexes2/7(FmHAM)
  [d_LLceHAM] -> Reflexes2/8(LceHAM)
  [d_LVceHAM] -> Reflexes2/9(VceHAM)
  [d_LFmRF] -> Reflexes2/10(FmRF)
  [d_LLceRF] -> Reflexes2/11(LceRF)
  [d_LVceRF] -> Reflexes2/12(VceRF)
  [d_LFmVAS] -> Reflexes2/13(FmVAS)
  [d_LLceVAS] -> Reflexes2/14(LceVAS)
  [d_LVceVAS] -> Reflexes2/15(VceVAS)
  [d_LFmBFSH] -> Reflexes2/16(FmBFSH)
  [d_LLceBFSH] -> Reflexes2/17(LceBFSH)
  [d_LVceBFSH] -> Reflexes2/18(VceBFSH)
  [d_LFmGAS] -> Reflexes2/19(FmGAS)
  [d_LLceGAS] -> Reflexes2/20(LceGAS)
  [d_LVceGAS] -> Reflexes2/21(VceGAS)
  [d_LFmSOL] -> Reflexes2/22(FmSOL)
  [d_LLceSOL] -> Reflexes2/23(LceSOL)
  [d_LVceSOL] -> Reflexes2/24(VceSOL)
  [d_LFmTA] -> Reflexes2/25(FmTA)
  [d_LLceTA] -> Reflexes2/26(LceTA)
  [d_LVceTA] -> Reflexes2/27(VceTA)
  [LActTA] -> Mux2/9
  [LActSOL] -> Mux2/8
  [LActGAS] -> Mux2/7
  [LActBFSH] -> Mux2/6
  [LActVAS] -> Mux2/5
  [LActRF] -> Mux2/4
  [LActHAM] -> Mux2/3
  [LActGLU] -> Mux2/2
  [LActHFL] -> Mux2/1
  Mux2/1 -> Reflexes2/28(Act)
  Reflexes2/1(Outport) -> [LExc_HFL_MN]
  Reflexes2/2(Outport1) -> [LExc_GLU_MN]
  Reflexes2/3(Outport2) -> [LExc_HAM_MN]
  Reflexes2/4(Outport3) -> [LExc_RF_MN]
  Reflexes2/5(Outport4) -> [LExc_VAS_MN]
  Reflexes2/6(Outport5) -> [LExc_BFSH_MN]
  Reflexes2/7(Outport6) -> [LExc_GAS_MN]
  Reflexes2/8(Outport7) -> [LExc_SOL_MN]
  Reflexes2/9(Outport8) -> [LExc_TA_MN]
  [d_RFmHFL] -> Reflexes1/4(FmHFL)
  [d_RFmBFSH] -> Reflexes1/16(FmBFSH)
  [d_RVceRF] -> Reflexes1/12(VceRF)
  [d_RVceBFSH] -> Reflexes1/18(VceBFSH)
  [d_RLceRF] -> Reflexes1/11(LceRF)
  [d_RFmRF] -> Reflexes1/10(FmRF)
  [d_RLceBFSH] -> Reflexes1/17(LceBFSH)
  [d_RLceVAS] -> Reflexes1/14(LceVAS)
  [d_RFmGAS] -> Reflexes1/19(FmGAS)
  [RActHAM] -> Mux3/3
  [RActGLU] -> Mux3/2
  [RActRF] -> Mux3/4
  [d_RVceTA] -> Reflexes1/27(VceTA)
  [d_RVceHFL] -> Reflexes1/6(VceHFL)
  [d_RLceHAM] -> Reflexes1/8(LceHAM)
  [d_RFmHAM] -> Reflexes1/7(FmHAM)
  [d_RLceHFL] -> Reflexes1/5(LceHFL)
  [RActBFSH] -> Mux3/6
  [RActVAS] -> Mux3/5
  [d_RVceGLU] -> Reflexes1/3(VceGLU)
  [d_RFmGLU] -> Reflexes1/1(FmGLU)
  [RActSOL] -> Mux3/8
  [RActTA] -> Mux3/9
  [d_RVceVAS] -> Reflexes1/15(VceVAS)
  [d_RLceTA] -> Reflexes1/26(LceTA)
  [d_RVceSOL] -> Reflexes1/24(VceSOL)
  [d_RVceGAS] -> Reflexes1/21(VceGAS)
  Mux3/1 -> Reflexes1/28(Act)
  [d_RFmVAS] -> Reflexes1/13(FmVAS)
  [d_RLceSOL] -> Reflexes1/23(LceSOL)
  [d_RFmTA] -> Reflexes1/25(FmTA)
  [d_RFmSOL] -> Reflexes1/22(FmSOL)
  [RActGAS] -> Mux3/7
  [d_RLceGLU] -> Reflexes1/2(LceGLU)
  [d_RLceGAS] -> Reflexes1/20(LceGAS)
  [d_RVceHAM] -> Reflexes1/9(VceHAM)
  [RActHFL] -> Mux3/1
  [LExc_RF_cpg] -> Sum9/1
  [LExc_VAS_cpg] -> Sum10/1
  [LExc_BFSH_cpg] -> Sum11/1
  [LExc_GAS_cpg] -> Sum12/1
  [LExc_SOL_cpg] -> Sum13/1
  [LExc_TA_cpg] -> Sum14/1
  Sum13/1 -> MN10/1(in)
  [RExc_RF_cpg] -> Sum23/1
  [RExc_GAS_cpg] -> Sum16/1
  [RExc_VAS_cpg] -> Sum6/1
  [RExc_SOL_cpg] -> Sum17/1
  [RExc_TA_cpg] -> Sum18/1
  [RExc_BFSH_cpg] -> Sum15/1
  Mux1/1 -> Saturation1/1
  Reflexes1/1(Outport) -> [RExc_HFL_MN]  "Exc HFL"
  Reflexes1/2(Outport1) -> [RExc_GLU_MN]  "Exc GLU"
  Reflexes1/9(Outport8) -> [RExc_TA_MN]  "Exc TA"
  Reflexes1/8(Outport7) -> [RExc_SOL_MN]  "Exc SOL"
  Reflexes1/7(Outport6) -> [RExc_GAS_MN]  "Exc GAS"
  Reflexes1/6(Outport5) -> [RExc_BFSH_MN]  "Exc BFSH"
  Reflexes1/5(Outport4) -> [RExc_VAS_MN]  "Exc VAS"
  Reflexes1/4(Outport3) -> [RExc_RF_MN]  "Exc RF"
  Reflexes1/3(Outport2) -> [RExc_HAM_MN]  "Exc HAM"
  [d_RStance] -> phi right/2(RStance)
  phi right/1(phi out) -> phi left3/2(In1), Central Pattern Generator/2(phi right)
  phi left3/1(phi out) -> phi right/1(In1), Central Pattern Generator/1(phi out)
  [d_LStance] -> phi left3/1(LStance)
  Sum18/1 -> MN/1(in)
  Sum17/1 -> MN1/1(in)
  Sum16/1 -> MN2/1(in)
  Sum15/1 -> MN3/1(in)
  Sum20/1 -> MN7/1(in)
  Sum6/1 -> MN4/1(in)
  Sum23/1 -> MN5/1(in)
  Sum22/1 -> MN6/1(in)
  Sum5/1 -> MN8/1(in)
  Sum1/1 -> MN17/1(in)
  Sum11/1 -> MN12/1(in)
  Sum3/1 -> MN16/1(in)
  Sum8/1 -> MN15/1(in)
  [d_theta] -> Balance Control System HAM/1(d_theta), Balance Control System GLU/1(d_theta), Balance Control System HFL/1(d_theta)
  [d_dtheta] -> Balance Control System HAM/2(d_dtheta), Balance Control System GLU/2(d_dtheta), Balance Control System HFL/2(d_dtheta)
  MN/1(out) -> Saturation44/1
  MN1/1(out) -> Saturation45/1
  MN3/1(out) -> Saturation47/1
  MN2/1(out) -> Saturation46/1
  MN4/1(out) -> Saturation48/1
  MN6/1(out) -> Saturation50/1
  MN7/1(out) -> Saturation51/1
  MN5/1(out) -> Saturation49/1
  MN8/1(out) -> Saturation52/1
  MN14/1(out) -> Saturation58/1
  MN13/1(out) -> Saturation57/1
  MN16/1(out) -> Saturation60/1
  MN17/1(out) -> Saturation61/1
  MN15/1(out) -> Saturation59/1
  MN9/1(out) -> Saturation53/1
  MN10/1(out) -> Saturation54/1
  MN11/1(out) -> Saturation55/1
  MN12/1(out) -> Saturation56/1
  Sum/1 -> Mux/1
  Sum2/1 -> Mux/2
  Sum4/1 -> Mux/3
  Sum7/1 -> Mux1/1
  Sum19/1 -> Mux1/2
  Sum21/1 -> Mux1/3
  Saturation50/1 -> Sum21/2  "ham"
  Saturation48/1 -> Mux1/5  "vas"
  Saturation52/1 -> Sum7/2  "hfl"
  Saturation44/1 -> Mux1/9  "ta"
  Saturation45/1 -> Mux1/8  "sol"
  Saturation47/1 -> Mux1/6  "bfsh"
  Saturation49/1 -> Mux1/4  "rf"
  Saturation51/1 -> Sum19/2  "glu"
  Saturation46/1 -> Mux1/7  "gas"
  Sum14/1 -> MN9/1(in)
  Sum12/1 -> MN11/1(in)
  Sum9/1 -> MN14/1(in)
  Sum10/1 -> MN13/1(in)
  [LExc_HFL_bal] -> Sum/1
  [LExc_GLU_bal] -> Sum2/1
  [LExc_HAM_bal] -> Sum4/1
  [RExc_HFL_bal] -> Sum7/1
  [RExc_HAM_bal] -> Sum21/1
  [RExc_GLU_bal] -> Sum19/1
  [LExc_HFL_cpg] -> Sum1/1
  [LExc_GLU_cpg] -> Sum3/1
  [LExc_HAM_cpg] -> Sum8/1
  [RExc_HAM_cpg] -> Sum22/1
  [RExc_GLU_cpg] -> Sum20/1
  [RExc_HFL_cpg] -> Sum5/1
  Product1/1 -> [RExc_HFL_bal]
  Product/1 -> [LExc_HFL_bal]
  Balance Control System GLU/1(ubalance) -> Product2/2, Product3/2
  Product2/1 -> [LExc_HAM_bal]
  Product3/1 -> [RExc_HAM_bal]
  Balance Control System HAM/1(ubalance) -> Product4/2, Product5/2
  Product5/1 -> [RExc_GLU_bal]
  Product4/1 -> [LExc_GLU_bal]
  [LExc_HFL_MN] -> Sum1/2
  [LExc_GLU_MN] -> Sum3/2
  [LExc_HAM_MN] -> Sum8/2
  [LExc_RF_MN] -> Sum9/2
  [LExc_VAS_MN] -> Sum10/2
  [LExc_BFSH_MN] -> Sum11/2
  [LExc_GAS_MN] -> Sum12/2
  [LExc_SOL_MN] -> Sum13/2
  [LExc_TA_MN] -> Sum14/2
  [RExc_TA_MN] -> Sum18/2
  [RExc_SOL_MN] -> Sum17/2
  [RExc_GAS_MN] -> Sum16/2
  [RExc_BFSH_MN] -> Sum15/2
  [RExc_VAS_MN] -> Sum6/2
  [RExc_RF_MN] -> Sum23/2
  [RExc_HAM_MN] -> Sum22/2
  [RExc_GLU_MN] -> Sum20/2
  [RExc_HFL_MN] -> Sum5/2
  Saturation61/1 -> Sum/2  "hfl"
  Saturation60/1 -> Sum2/2  "glu"
  Saturation59/1 -> Sum4/2  "ham"
  Saturation58/1 -> Mux/4  "rf"
  Saturation57/1 -> Mux/5  "vas"
  Saturation56/1 -> Mux/6  "bfsh"
  Saturation55/1 -> Mux/7  "gas"
  Saturation54/1 -> Mux/8  "sol"
  Saturation53/1 -> Mux/9  "ta"

== system nms_sim_2D_cost/Cost ==
  note: Cost
  ACT : Subsystem
  Clock3 : Clock
  Compare To Constant4 : simulink/Logic and Bit Operations/Compare To Constant  relop=<  const=0.25*sub_height  OutDataTypeStr=boolean
  Gain : Gain  Gain=.5
  Gain1 : Gain  Gain=.5
  Gain2 : Gain  Gain=.5
  Mux17 : Mux  Inputs=6
  SS_dist : Subsystem  TreatAsAtomicUnit=on
  Selector{7,9..10,28} (4 alike) : Selector  InputPortWidth=3  IndexOptions=Index vector (dialog)  Indices=2  OutputSizes=1
  Selector{12..16,18} (6 alike) : Selector  InputPortWidth=3  IndexOptions=Index vector (dialog)  Indices=[1 2]  OutputSizes=1
  Step Counter : Subsystem
  Stop Simulation1 : Stop
  Stop Simulation3 : Stop
  Sum : Sum  Inputs=|++
  Sum1 : Sum  Inputs=|+-
  Sum2 : Sum  Inputs=|++
  Sum3 : Sum  Inputs=|++
  To Workspace1 : ToWorkspace  VariableName=tEnd  SaveFormat=Timeseries  SampleTime=-1
      settings: MaxDataPoints=1
  To Workspace2 : ToWorkspace  VariableName=xHAT_end  SaveFormat=Timeseries  SampleTime=-1
      settings: MaxDataPoints=1
  To Workspace3 : ToWorkspace  VariableName=flag_fall  SaveFormat=Timeseries  SampleTime=-1
      settings: MaxDataPoints=1
  To Workspace5 : ToWorkspace  VariableName=flag  SaveFormat=Timeseries  SampleTime=-1
      settings: MaxDataPoints=1
  calculate ObjFn : Subsystem  TreatAsAtomicUnit=on
  check steady state : Subsystem
  flight : Subsystem
  hipM1 : Selector  InputPortWidth=3  IndexOptions=Index vector (dialog)  Indices=1  OutputSizes=1
  hipM2 : Selector  InputPortWidth=3  IndexOptions=Index vector (dialog)  Indices=1  OutputSizes=1
  joint overextension : Subsystem
  nStep start : Subsystem  TreatAsAtomicUnit=on
  wires:
  [xyzHAT1] -> Selector13/1
  [xyzLFoot2] -> Selector15/1
  Selector15/1 -> Mux17/5
  Mux17/1 -> check steady state/1(p)
  Selector12/1 -> Mux17/1
  [xyzLShank1] -> Selector16/1
  [xyzRShank1] -> Selector18/1
  [xyzHAT2] -> Selector14/1
  Selector14/1 -> Mux17/4
  Selector13/1 -> Mux17/3
  [xyzRFoot2] -> Selector12/1
  [RStance] -> Step Counter/1(RStance)  "RStance"
  Selector16/1 -> Mux17/6
  Selector18/1 -> Mux17/2
  [LStance] -> SS_dist/Trigger, Step Counter/2(LStance)  "LStance"
  check steady state/2(SS_dist) -> SS_dist/1(SS_dist)
  nStep start/1(nStep_start) -> calculate ObjFn/2(nStep_start)
  Step Counter/1(nStep) -> nStep start/1(nStep), calculate ObjFn/1(nStep), check steady state/2(nStep)
  calculate ObjFn/1(stop) -> To Workspace5/1, Stop Simulation1/1
  [xyzHAT] -> hipM2/1
  ACT/1(ACT) -> calculate ObjFn/3(ACT)
  Clock3/1 -> To Workspace1/1, calculate ObjFn/7(t [s])
  check steady state/1(SS) -> nStep start/Trigger, calculate ObjFn/Enable
  joint overextension/1(pain) -> calculate ObjFn/4(pain)
  [xyzHAT] -> hipM1/1
  hipM2/1 -> Sum/1
  hipM1/1 -> Sum/2
  Sum/1 -> Gain/1
  Gain/1 -> calculate ObjFn/6(x), To Workspace2/1
  [xyzLShank1] -> Selector9/1
  [xyzRShank1] -> Selector10/1
  Selector9/1 -> Sum2/1
  Selector10/1 -> Sum2/2
  Sum2/1 -> Gain1/1
  Gain1/1 -> Sum1/2
  Sum1/1 -> Compare To Constant4/1
  Gain2/1 -> Sum1/1
  Sum3/1 -> Gain2/1
  Selector7/1 -> Sum3/2
  Selector28/1 -> Sum3/1
  [xyzRHip] -> Selector7/1
  [xyzLHip] -> Selector28/1
  Compare To Constant4/1 -> To Workspace3/1, Stop Simulation3/1
  flight/1(flight) -> calculate ObjFn/5(flight)
